simulink model "DSP_Simulink"  (R2023a)
settings: Solver=FixedStepAuto  StartTime=0.0  StopTime=10.0  RelTol=1e-3
undefined symbols (not defined in the file): Altitude, DSP_final_pro, Latitude, Longitude, STATE, State_change, STATIONARY_NODE, Timestamp
libraries: androidcommunicationlib x8, androiduilib x7, simulink x6, androidaudiovideolib x4, androidsensorlib x3
settings Model: Creator=visha  LastModifiedBy=visha
settings OptimizationCC: EnhancedBackFolding=on  PassReuseOutputArgsAs=Individual arguments  ZeroExternalMemoryAtStartup=off  ZeroInternalMemoryAtStartup=off  MaxStackSize=64  OptimizeBlockOrder=speed  DifferentSizesBufferReuse=on  OptimizationCustomize=off  EfficientTunableParamExpr=on
settings DebuggingCC: ParameterTunabilityLossMsg=error
settings HardwareCC: ProdBitPerPointer=32  ProdBitPerSizeT=32  ProdBitPerPtrDiffT=32  ProdLargestAtomicInteger=Long  ProdLargestAtomicFloat=Double  ProdWordSize=32  ProdHWDeviceType=ARM Compatible->ARM Cortex
settings SFSimCC: MATLABDynamicMemAlloc=off
settings RTWCC: Description=Embedded Coder  SystemTargetFile=ert.tlc  HardwareBoard=Android Device  TLCOptions="-aInlineSetEventsForThisBaseRateFcn=TLC_FALSE -aSuppressMultiTaskScheduler=TLC_FALSE  -aRateBasedStepFcn=0"  TemplateMakefile=ert_default_tmf  RTWVerbose=off  Toolchain=Android SDK/NDK Tools
settings CodeAppCC: ForceParamTrailComments=on  IgnoreCustomStorageClasses=off  OperatorAnnotations=on  SimulinkDataObjDesc=on  SFDataObjDesc=on  InsertBlockDesc=on

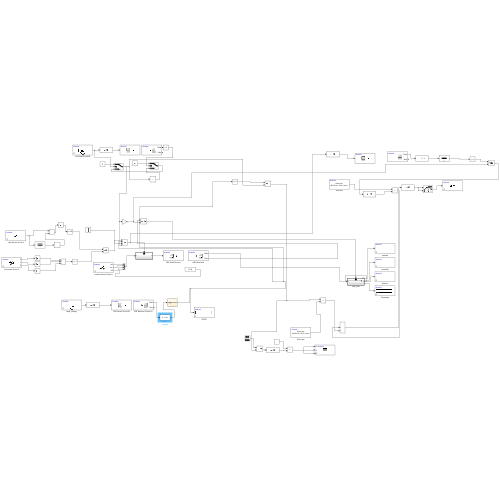
[thumbnail: Simulink's stored preview of the top-level diagram]
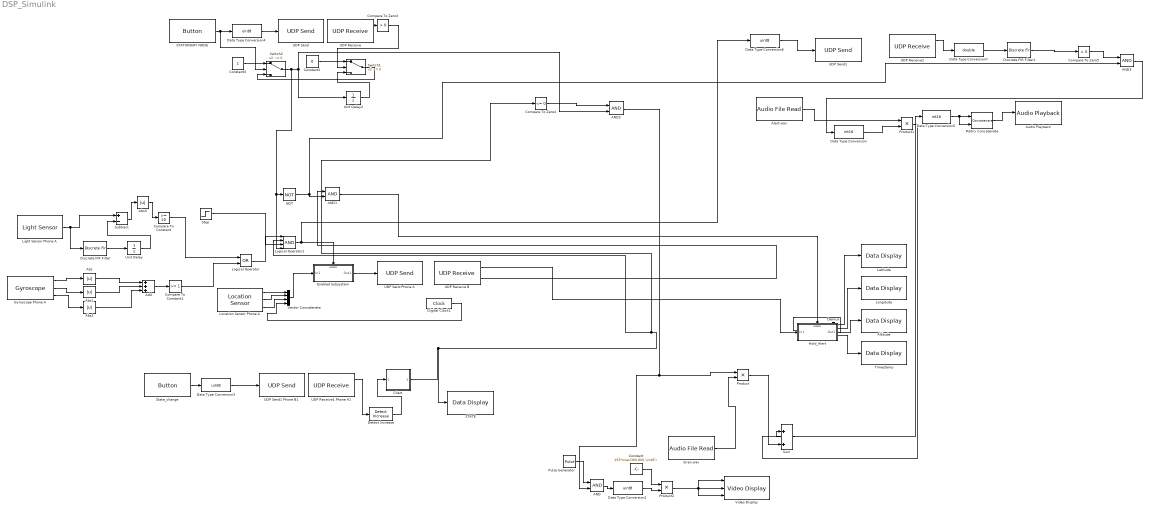
== system DSP_Simulink ==
  AND{,1..3} (4 alike) : Logic  AllPortsSameDT=off  OutDataTypeStr=boolean
  Abs{,1..3} (4 alike) : Abs  SaturateOnIntegerOverflow=off
  Add : Sum  Inputs=+++
  Alert.wav : androidaudiovideolib/Audio File Read  FileName=C:\simwork\Alert.wav  FrameSize=441
  Altitude : androiduilib/Data Display  DataDisplayId=DSP_final_pro/Altitude  Format=Float  Precision=6  SimulateUsing=Code generation  blockPlatform=Android
  Audio Playback : androidaudiovideolib/Audio Playback  SampleFreq=44100  AudioSamplingFreq=44100  SampleTime=0.1  DeviceStr=0  QueueDuration=0  BlockPlatform=Android
  Chart : Stateflow chart  TreatAsAtomicUnit=on
  Compare To Constant : simulink/Logic and Bit Operations/Compare To Constant  relop=>=  const=20  OutDataTypeStr=boolean
  Compare To Constant1 : simulink/Logic and Bit Operations/Compare To Constant  relop=>=  const=1  OutDataTypeStr=boolean
  Compare To Zero3 : simulink/Logic and Bit Operations/Compare To Zero  relop=>  OutDataTypeStr=boolean
  Compare To Zero4 : simulink/Logic and Bit Operations/Compare To Zero  relop=<=  OutDataTypeStr=boolean
  Compare To Zero5 : simulink/Logic and Bit Operations/Compare To Zero  relop=>  OutDataTypeStr=boolean
  Constant : Constant  Value=255*ones(360,800,'uint8')
  Constant2 : Constant  Value=0
  Constant3 : Constant
  Data Type Conversion : DataTypeConversion  OutDataTypeStr=int16  SaturateOnIntegerOverflow=off  RndMeth=Floor
  Data Type Conversion{2..4,6} (4 alike) : DataTypeConversion  OutDataTypeStr=uint8  SaturateOnIntegerOverflow=off  RndMeth=Floor
  Data Type Conversion5 : DataTypeConversion  OutDataTypeStr=int16  SaturateOnIntegerOverflow=off  RndMeth=Floor
  Data Type Conversion7 : DataTypeConversion  OutDataTypeStr=double  SaturateOnIntegerOverflow=off  RndMeth=Floor
  Demux : Demux
  Detect Increase : simulink/Logic and Bit Operations/Detect Increase  vinit=0.0  OutDataTypeStr=boolean
  Digital Clock1 : DigitalClock
  Discrete FIR Filter : DiscreteFir  Coefficients=ones(1,20)/20
  Discrete FIR Filter1 : DiscreteFir  Coefficients=ones(1,10)
  Enabled Subsystem : Subsystem  TreatAsAtomicUnit=on
  Gyroscope Phone A : androidsensorlib/Gyroscope  OutputVector=off  SampleTime=0.1  BlockPlatform=Android
  Hold_Alert : Subsystem  TreatAsAtomicUnit=on
  Latitude : androiduilib/Data Display  DataDisplayId=DSP_final_pro/Latitude  Format=Float  Precision=6  SimulateUsing=Code generation  blockPlatform=Android
  Light Sensor Phone A : androidsensorlib/Light Sensor  SampleTime=0.1  BlockPlatform=Android
  Location Sensor Phone A : androidsensorlib/Location Sensor  OutputVector=off  SampleTime=0.1  BlockPlatform=Android
  Logical Operator : Logic  Operator=OR  AllPortsSameDT=off  OutDataTypeStr=boolean
  Logical Operator1 : Logic  Inputs=4  AllPortsSameDT=off  OutDataTypeStr=boolean
  Longitude : androiduilib/Data Display  DataDisplayId=DSP_final_pro/Longitude  Format=Float  Precision=6  SimulateUsing=Code generation  blockPlatform=Android
  Matrix Concatenate : Concatenate  Mode=Multidimensional array  ConcatenateDimension=2
  NOT : Logic  Operator=NOT  IconShape=distinctive  AllPortsSameDT=off  OutDataTypeStr=boolean
  Product : Product
  Product1 : Product
  Product2 : Product
  Pulse Generator : DiscretePulseGenerator  Period=4  PulseWidth=2  SampleTime=0.25
  STATE : androiduilib/Data Display  DataDisplayId=DSP_final_pro/STATE  Format=Float  Precision=6  SimulateUsing=Code generation  blockPlatform=Android
  STATIONARY NODE : androiduilib/Button  ButtonState=Not pressed  ButtonId=DSP_final_pro/STATIONARY_NODE  State=off  SampleTime=0.1  BlockPlatform=Android
  Siren.wav : androidaudiovideolib/Audio File Read  FileName=C:\simwork\Siren.wav  FrameSize=441
  State_change : androiduilib/Button  ButtonState=Not pressed  ButtonId=DSP_final_pro/State_change  State=off  SampleTime=0.1  BlockPlatform=Android
  Step : Step  Time=5  SampleTime=0.1
  Subtract : Sum  Inputs=+-
  Sum : Sum  Inputs=|++
  Switch1 : Switch  Criteria=u2 ~= 0  SaturateOnIntegerOverflow=off  InputSameDT=off
  Switch2 : Switch  Criteria=u2 ~= 0  SaturateOnIntegerOverflow=off  InputSameDT=off
  Timestamp : androiduilib/Data Display  DataDisplayId=DSP_final_pro/Timestamp  Format=Float  Precision=6  SimulateUsing=Code generation  blockPlatform=Android
  UDP Receive : androidcommunicationlib/UDP Receive  localURL='0.0.0.0'  localPort=25004  remoteURL='0.0.0.0'  remotePort=-1  recvBufferSize=8192  signalDatatype=uint8  dims=1  isVarSize=off  showBlockingTime=off  blockingTime=0  sampletime=0.01  blockPlatform=Android
  UDP Receive B : androidcommunicationlib/UDP Receive  localURL='0.0.0.0'  localPort=25000  remoteURL='0.0.0.0'  remotePort=-1  recvBufferSize=8192  signalDatatype=double  dims=4  isVarSize=off  showBlockingTime=off  blockingTime=0  sampletime=0.01  blockPlatform=Android
  UDP Receive1 : androidcommunicationlib/UDP Receive  localURL='0.0.0.0'  localPort=25005  remoteURL='0.0.0.0'  remotePort=-1  recvBufferSize=8192  signalDatatype=uint8  dims=1  isVarSize=off  showBlockingTime=off  blockingTime=0  sampletime=0.01  blockPlatform=Android
  UDP Receive1 Phone A1 : androidcommunicationlib/UDP Receive  localURL='0.0.0.0'  localPort=25002  remoteURL='0.0.0.0'  remotePort=-1  recvBufferSize=8192  signalDatatype=boolean  dims=1  isVarSize=off  showBlockingTime=off  blockingTime=0  sampletime=0.1  blockPlatform=Android
  UDP Send : androidcommunicationlib/UDP Send  remoteURL='10.7.19.244'  remotePort=25004  localURL='0.0.0.0'  localPortSource=Automatically determine  localPort=-1  sampletime=-1  blockPlatform=Android  separateLengthPort=0
  UDP Send Phone A : androidcommunicationlib/UDP Send  remoteURL='10.7.19.244'  remotePort=25000  localURL='0.0.0.0'  localPortSource=Automatically determine  localPort=-1  sampletime=-1  blockPlatform=Android  separateLengthPort=0
  UDP Send1 : androidcommunicationlib/UDP Send  remoteURL='10.7.19.244'  remotePort=25005  localURL='0.0.0.0'  localPortSource=Automatically determine  localPort=-1  sampletime=-1  blockPlatform=Android  separateLengthPort=0
  UDP Send1 Phone B1 : androidcommunicationlib/UDP Send  remoteURL='10.7.19.244'  remotePort=25002  localURL='0.0.0.0'  localPortSource=Automatically determine  localPort=-1  sampletime=-1  blockPlatform=Android  separateLengthPort=0
  Unit Delay : UnitDelay  SampleTime=-1  HasFrameUpgradeWarning=on
  Unit Delay2 : UnitDelay  SampleTime=-1  HasFrameUpgradeWarning=on
  Vector Concatenate : Concatenate  NumInputs=4
  Video Display : androidaudiovideolib/Video Display  BlockPlatform=Android
  wires:
  Abs3/1 -> Compare To Constant/1
  Subtract/1 -> Abs3/1
  Discrete FIR Filter1/1 -> Compare To Zero5/1
  AND2/1 -> AND/2, Product/1
  Compare To Zero5/1 -> AND3/1
  Product2/1 -> Video Display/3, Video Display/2, Video Display/1
  Switch1/1 -> Switch2/3
  UDP Receive/1 -> Compare To Zero3/1
  Unit Delay2/1 -> Switch1/3
  NOT/1 -> AND3/2, AND1/2
  Constant2/1 -> Switch1/1
  Data Type Conversion4/1 -> UDP Send/1
  Data Type Conversion5/1 -> Matrix Concatenate/2, Matrix Concatenate/1
  Constant3/1 -> Switch2/1
  Data Type Conversion6/1 -> UDP Send1/1
  Matrix Concatenate/1 -> Audio Playback/1
  UDP Receive1/1 -> Data Type Conversion7/1
  AND1/1 -> Hold_Alert/Enable
  UDP Receive1 Phone A1/1 -> Detect Increase/1
  Discrete FIR Filter/1 -> Unit Delay/1
  State_change/1 -> Data Type Conversion3/1
  Detect Increase/1 -> Chart/1(toggle)
  UDP Receive B/1 -> Hold_Alert/1(In1)
  Gyroscope Phone A/2 -> Abs1/1
  Data Type Conversion/1 -> Product1/2
  Unit Delay/1 -> Subtract/2
  Constant/1 -> Product2/1
  Add/1 -> Compare To Constant1/1
  Logical Operator1/1 -> Data Type Conversion6/1, Enabled Subsystem/Enable
  Compare To Zero4/1 -> AND2/1
  Compare To Constant/1 -> Logical Operator/1
  Light Sensor Phone A/1 -> Discrete FIR Filter/1, Subtract/1
  STATIONARY NODE/1 -> Switch2/2, Data Type Conversion4/1
  Pulse Generator/1 -> AND/1
  Abs2/1 -> Add/3
  Switch2/1 -> NOT/1, Logical Operator1/4, AND2/2, Unit Delay2/1
  Vector Concatenate/1 -> Enabled Subsystem/1(In1)
  Demux/3 -> Altitude/1
  Siren.wav/1 -> Product/2
  Enabled Subsystem/1(Out1) -> UDP Send Phone A/1
  Product/1 -> Sum/2
  Demux/4 -> Timestamp/1
  Chart/1(is_armed) -> Logical Operator1/2, Compare To Zero4/1, STATE/1
  Demux/1 -> Latitude/1
  Abs/1 -> Add/1
  Gyroscope Phone A/1 -> Abs/1
  Product1/1 -> Sum/1
  Digital Clock1/1 -> Vector Concatenate/4
  Alert.wav/1 -> Product1/1
  Data Type Conversion3/1 -> UDP Send1 Phone B1/1
  Location Sensor Phone A/2 -> Vector Concatenate/2
  Step/1 -> Logical Operator1/3
  Location Sensor Phone A/1 -> Vector Concatenate/1
  Abs1/1 -> Add/2
  Location Sensor Phone A/3 -> Vector Concatenate/3
  Compare To Constant1/1 -> Logical Operator/2
  Sum/1 -> Data Type Conversion5/1
  Gyroscope Phone A/3 -> Abs2/1
  UDP Receive B/2 -> AND1/1
  Demux/2 -> Longitude/1
  Data Type Conversion2/1 -> Product2/2
  Hold_Alert/1(Out1) -> Demux/1
  Compare To Zero3/1 -> Switch1/2
  AND/1 -> Data Type Conversion2/1
  Logical Operator/1 -> Logical Operator1/1
  Data Type Conversion7/1 -> Discrete FIR Filter1/1
  AND3/1 -> Data Type Conversion/1

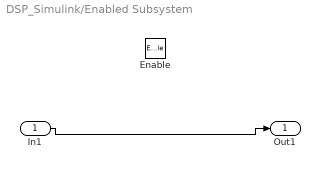
== system DSP_Simulink/Enabled Subsystem ==
  In1 : Inport
  Enable : EnablePort
  Out1 : Outport
  wires:
  In1/1 -> Out1/1

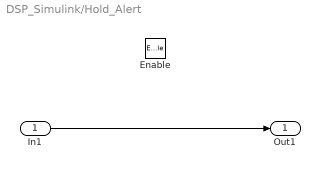
== system DSP_Simulink/Hold_Alert ==
  In1 : Inport
  Enable : EnablePort
  Out1 : Outport
  wires:
  In1/1 -> Out1/1

== stateflow chart DSP_Simulink/Chart ==
  state DISARMED
    entry: is_armed = 0;
  state ARMED
    entry: is_armed = 1;
  (default) -> ARMED
  ARMED -> DISARMED : [toggle == 1]
  DISARMED -> ARMED : [toggle == 1]
  data: is_armed output; toggle input
